simulink model "bms_can_unpack"  (R2026b)
settings: Solver=VariableStepAuto
undefined symbols (not defined in the file or in its folder): Ts
libraries: simulink x16, svdutilitieslib x7
settings Model: Creator=aomar  LastModifiedBy=aomar

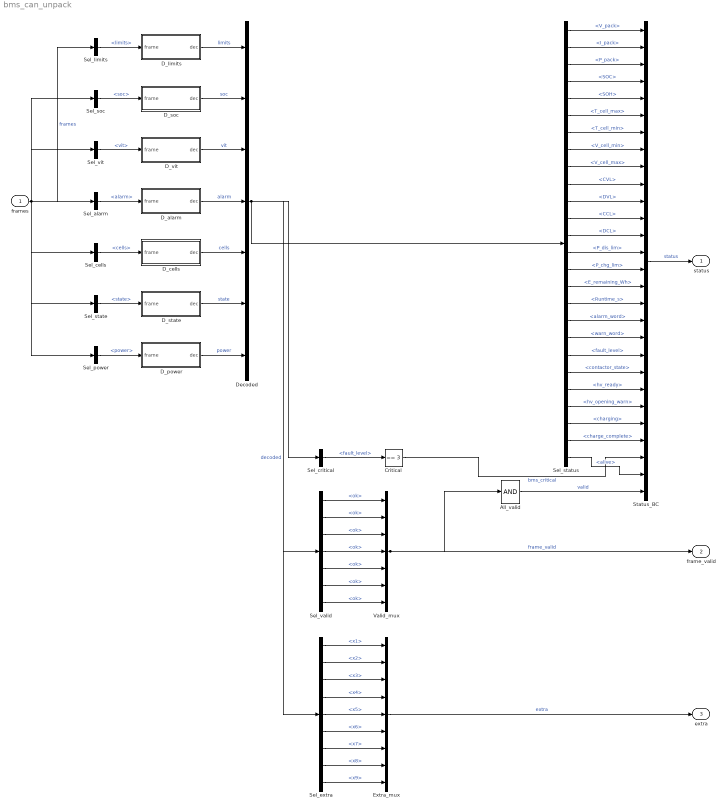
== system bms_can_unpack ==
  frames : Inport  OutDataTypeStr=Bus: Bus_Can1_Bms  SampleTime=Ts.hk
  All_valid : Logic  Inputs=1  AllPortsSameDT=off  OutDataTypeStr=boolean
  Critical : simulink/Logic and Bit Operations/Compare To Constant  relop===  const=3  OutDataTypeStr=boolean
  D_alarm : Subsystem
  D_cells : Subsystem
  D_limits : Subsystem
  D_power : Subsystem
  D_soc : Subsystem
  D_state : Subsystem
  D_vit : Subsystem
  Decoded : BusCreator  Inputs=7
  Extra_mux : Mux  Inputs=9
  Sel_alarm : BusSelector  OutputSignals=alarm
  Sel_cells : BusSelector  OutputSignals=cells
  Sel_critical : BusSelector  OutputSignals=state.fault_level
  Sel_extra : BusSelector  OutputSignals=vit.x1,vit.x2,soc.x3,power.x4,soc.x5,state.x6,state.x7,state.x8,state.x9
  Sel_limits : BusSelector  OutputSignals=limits
  Sel_power : BusSelector  OutputSignals=power
  Sel_soc : BusSelector  OutputSignals=soc
  Sel_state : BusSelector  OutputSignals=state
  Sel_status : BusSelector  OutputSignals=vit.V_pack,vit.I_pack,power.P_pack,soc.SOC,soc.SOH,cells.T_cell_max,cells.T_cell_min,cells.V_cell_min,cells.V_cell_max,limits.CVL,limits.DVL,limits.CCL,limits.DCL,power.P_dis_lim,power.P_chg_lim,state.E_remaining_Wh,state.Runtime_s,alarm.alarm_word,alarm.warn_word,state.fault_level,state.contactor_state,state.hv_ready,state.hv_opening_warn,state.charging,state.charge_complete,state.alive
  Sel_valid : BusSelector  OutputSignals=limits.ok,soc.ok,vit.ok,alarm.ok,cells.ok,state.ok,power.ok
  Sel_vit : BusSelector  OutputSignals=vit
  Status_BC : BusCreator  Inputs=28  OutDataTypeStr=Bus: Bus_BmsStatus  NonVirtualBus=on
      settings: InheritFromInputs=off
  Valid_mux : Mux  Inputs=7
  status : Outport  OutDataTypeStr=Bus: Bus_BmsStatus
  frame_valid : Outport  Port=2  OutDataTypeStr=boolean
  extra : Outport  Port=3  OutDataTypeStr=single
  wires:
  frames/1 -> Sel_limits/1, Sel_power/1, Sel_soc/1, Sel_state/1, Sel_vit/1, Sel_cells/1, Sel_alarm/1  "frames"
  Sel_limits/1 -> D_limits/1(frame)  "<limits>"
  Sel_soc/1 -> D_soc/1(frame)  "<soc>"
  Sel_vit/1 -> D_vit/1(frame)  "<vit>"
  Sel_alarm/1 -> D_alarm/1(frame)  "<alarm>"
  Sel_cells/1 -> D_cells/1(frame)  "<cells>"
  Sel_state/1 -> D_state/1(frame)  "<state>"
  Sel_power/1 -> D_power/1(frame)  "<power>"
  D_limits/1(dec) -> Decoded/1  "limits"
  D_soc/1(dec) -> Decoded/2  "soc"
  D_vit/1(dec) -> Decoded/3  "vit"
  D_alarm/1(dec) -> Decoded/4  "alarm"
  D_cells/1(dec) -> Decoded/5  "cells"
  D_state/1(dec) -> Decoded/6  "state"
  D_power/1(dec) -> Decoded/7  "power"
  Decoded/1 -> Sel_extra/1, Sel_valid/1, Sel_critical/1, Sel_status/1  "decoded"
  Sel_critical/1 -> Critical/1  "<fault_level>"
  Sel_valid/1 -> Valid_mux/1  "<ok>"
  Sel_valid/2 -> Valid_mux/2  "<ok>"
  Sel_valid/3 -> Valid_mux/3  "<ok>"
  Sel_valid/4 -> Valid_mux/4  "<ok>"
  Sel_valid/5 -> Valid_mux/5  "<ok>"
  Sel_valid/6 -> Valid_mux/6  "<ok>"
  Sel_valid/7 -> Valid_mux/7  "<ok>"
  Sel_extra/1 -> Extra_mux/1  "<x1>"
  Sel_extra/2 -> Extra_mux/2  "<x2>"
  Sel_extra/3 -> Extra_mux/3  "<x3>"
  Sel_extra/4 -> Extra_mux/4  "<x4>"
  Sel_extra/5 -> Extra_mux/5  "<x5>"
  Sel_extra/6 -> Extra_mux/6  "<x6>"
  Sel_extra/7 -> Extra_mux/7  "<x7>"
  Sel_extra/8 -> Extra_mux/8  "<x8>"
  Sel_extra/9 -> Extra_mux/9  "<x9>"
  Valid_mux/1 -> All_valid/1, frame_valid/1  "frame_valid"
  Extra_mux/1 -> extra/1  "extra"
  Critical/1 -> Status_BC/26  "bms_critical"
  All_valid/1 -> Status_BC/28  "valid"
  Sel_status/1 -> Status_BC/1  "<V_pack>"
  Sel_status/2 -> Status_BC/2  "<I_pack>"
  Sel_status/3 -> Status_BC/3  "<P_pack>"
  Sel_status/4 -> Status_BC/4  "<SOC>"
  Sel_status/5 -> Status_BC/5  "<SOH>"
  Sel_status/6 -> Status_BC/6  "<T_cell_max>"
  Sel_status/7 -> Status_BC/7  "<T_cell_min>"
  Sel_status/8 -> Status_BC/8  "<V_cell_min>"
  Sel_status/9 -> Status_BC/9  "<V_cell_max>"
  Sel_status/10 -> Status_BC/10  "<CVL>"
  Sel_status/11 -> Status_BC/11  "<DVL>"
  Sel_status/12 -> Status_BC/12  "<CCL>"
  Sel_status/13 -> Status_BC/13  "<DCL>"
  Sel_status/14 -> Status_BC/14  "<P_dis_lim>"
  Sel_status/15 -> Status_BC/15  "<P_chg_lim>"
  Sel_status/16 -> Status_BC/16  "<E_remaining_Wh>"
  Sel_status/17 -> Status_BC/17  "<Runtime_s>"
  Sel_status/18 -> Status_BC/18  "<alarm_word>"
  Sel_status/19 -> Status_BC/19  "<warn_word>"
  Sel_status/20 -> Status_BC/20  "<fault_level>"
  Sel_status/21 -> Status_BC/21  "<contactor_state>"
  Sel_status/22 -> Status_BC/22  "<hv_ready>"
  Sel_status/23 -> Status_BC/23  "<hv_opening_warn>"
  Sel_status/24 -> Status_BC/24  "<charging>"
  Sel_status/25 -> Status_BC/25  "<charge_complete>"
  Sel_status/26 -> Status_BC/27  "<alive>"
  Status_BC/1 -> status/1  "status"

== system bms_can_unpack/D_alarm ==
  frame_id : Inport  PortName=frame  Element=id
  frame_valid : Inport  PortName=frame  Element=valid
  frame_data : Inport  PortName=frame  Element=data
  Decode : Subsystem  TreatAsAtomicUnit=on
  Frame_ok : Logic  AllPortsSameDT=off  OutDataTypeStr=boolean
  ID_match : simulink/Logic and Bit Operations/Compare To Constant  relop===  const=858  OutDataTypeStr=boolean
  dec_ok : Outport  PortName=dec  Element=ok
  dec_alarm_word : Outport  PortName=dec  Element=alarm_word
  dec_warn_word : Outport  PortName=dec  Element=warn_word
  wires:
  frame_id/1 -> ID_match/1  "id"
  ID_match/1 -> Frame_ok/1  "id_match"
  frame_valid/1 -> Frame_ok/2  "valid"
  Frame_ok/1 -> dec_ok/1, Decode/Enable  "frame_ok"
  frame_data/1 -> Decode/1(data)  "data"
  Decode/1(alarm_word) -> dec_alarm_word/1  "alarm_word"
  Decode/2(warn_word) -> dec_warn_word/1  "warn_word"

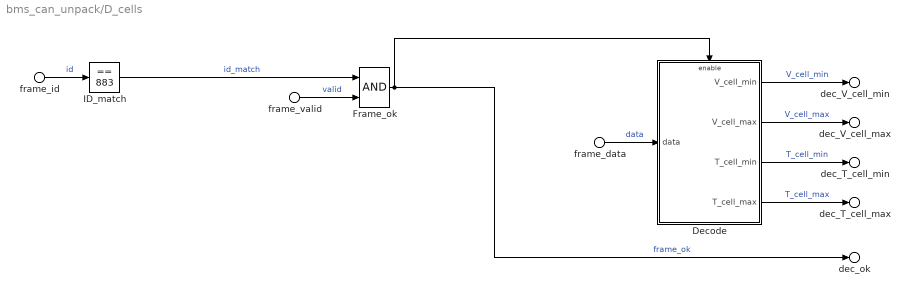
== system bms_can_unpack/D_cells ==
  frame_id : Inport  PortName=frame  Element=id
  frame_valid : Inport  PortName=frame  Element=valid
  frame_data : Inport  PortName=frame  Element=data
  Decode : Subsystem  TreatAsAtomicUnit=on
  Frame_ok : Logic  AllPortsSameDT=off  OutDataTypeStr=boolean
  ID_match : simulink/Logic and Bit Operations/Compare To Constant  relop===  const=883  OutDataTypeStr=boolean
  dec_ok : Outport  PortName=dec  Element=ok
  dec_V_cell_min : Outport  PortName=dec  Element=V_cell_min
  dec_V_cell_max : Outport  PortName=dec  Element=V_cell_max
  dec_T_cell_min : Outport  PortName=dec  Element=T_cell_min
  dec_T_cell_max : Outport  PortName=dec  Element=T_cell_max
  wires:
  frame_id/1 -> ID_match/1  "id"
  ID_match/1 -> Frame_ok/1  "id_match"
  frame_valid/1 -> Frame_ok/2  "valid"
  Frame_ok/1 -> dec_ok/1, Decode/Enable  "frame_ok"
  frame_data/1 -> Decode/1(data)  "data"
  Decode/1(V_cell_min) -> dec_V_cell_min/1  "V_cell_min"
  Decode/2(V_cell_max) -> dec_V_cell_max/1  "V_cell_max"
  Decode/3(T_cell_min) -> dec_T_cell_min/1  "T_cell_min"
  Decode/4(T_cell_max) -> dec_T_cell_max/1  "T_cell_max"

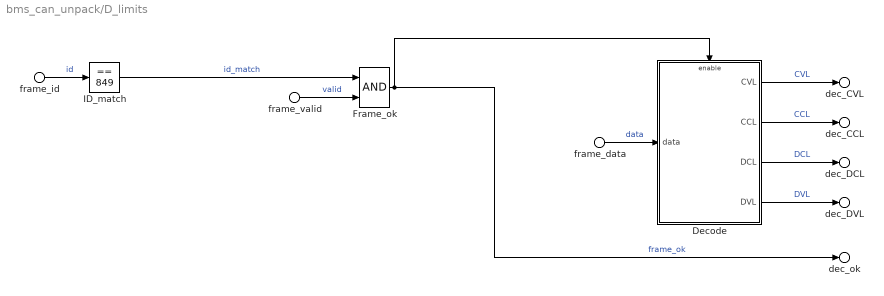
== system bms_can_unpack/D_limits ==
  frame_id : Inport  PortName=frame  Element=id
  frame_valid : Inport  PortName=frame  Element=valid
  frame_data : Inport  PortName=frame  Element=data
  Decode : Subsystem  TreatAsAtomicUnit=on
  Frame_ok : Logic  AllPortsSameDT=off  OutDataTypeStr=boolean
  ID_match : simulink/Logic and Bit Operations/Compare To Constant  relop===  const=849  OutDataTypeStr=boolean
  dec_ok : Outport  PortName=dec  Element=ok
  dec_CVL : Outport  PortName=dec  Element=CVL
  dec_CCL : Outport  PortName=dec  Element=CCL
  dec_DCL : Outport  PortName=dec  Element=DCL
  dec_DVL : Outport  PortName=dec  Element=DVL
  wires:
  frame_id/1 -> ID_match/1  "id"
  ID_match/1 -> Frame_ok/1  "id_match"
  frame_valid/1 -> Frame_ok/2  "valid"
  Frame_ok/1 -> dec_ok/1, Decode/Enable  "frame_ok"
  frame_data/1 -> Decode/1(data)  "data"
  Decode/1(CVL) -> dec_CVL/1  "CVL"
  Decode/2(CCL) -> dec_CCL/1  "CCL"
  Decode/3(DCL) -> dec_DCL/1  "DCL"
  Decode/4(DVL) -> dec_DVL/1  "DVL"

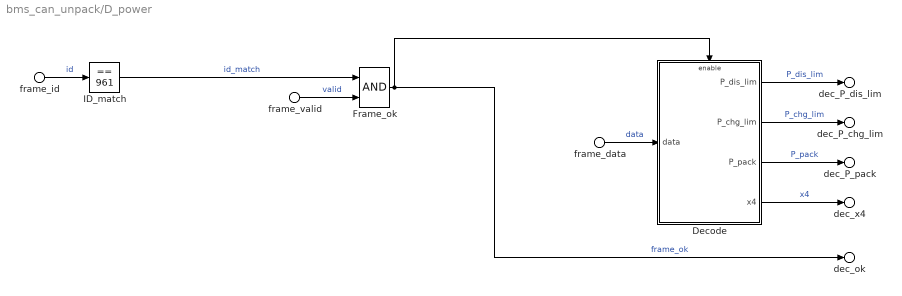
== system bms_can_unpack/D_power ==
  frame_id : Inport  PortName=frame  Element=id
  frame_valid : Inport  PortName=frame  Element=valid
  frame_data : Inport  PortName=frame  Element=data
  Decode : Subsystem  TreatAsAtomicUnit=on
  Frame_ok : Logic  AllPortsSameDT=off  OutDataTypeStr=boolean
  ID_match : simulink/Logic and Bit Operations/Compare To Constant  relop===  const=961  OutDataTypeStr=boolean
  dec_ok : Outport  PortName=dec  Element=ok
  dec_P_dis_lim : Outport  PortName=dec  Element=P_dis_lim
  dec_P_chg_lim : Outport  PortName=dec  Element=P_chg_lim
  dec_P_pack : Outport  PortName=dec  Element=P_pack
  dec_x4 : Outport  PortName=dec  Element=x4
  wires:
  frame_id/1 -> ID_match/1  "id"
  ID_match/1 -> Frame_ok/1  "id_match"
  frame_valid/1 -> Frame_ok/2  "valid"
  Frame_ok/1 -> dec_ok/1, Decode/Enable  "frame_ok"
  frame_data/1 -> Decode/1(data)  "data"
  Decode/1(P_dis_lim) -> dec_P_dis_lim/1  "P_dis_lim"
  Decode/2(P_chg_lim) -> dec_P_chg_lim/1  "P_chg_lim"
  Decode/3(P_pack) -> dec_P_pack/1  "P_pack"
  Decode/4(x4) -> dec_x4/1  "x4"

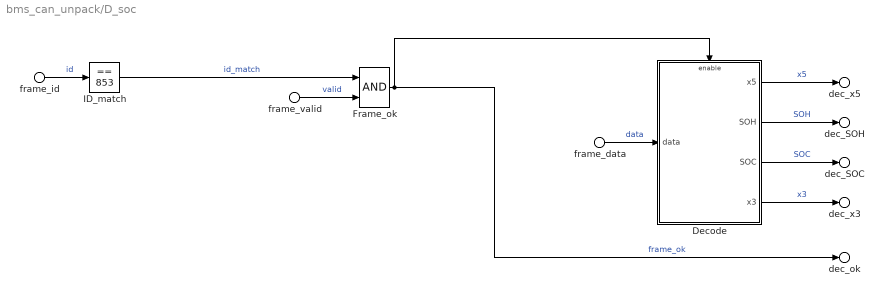
== system bms_can_unpack/D_soc ==
  frame_id : Inport  PortName=frame  Element=id
  frame_valid : Inport  PortName=frame  Element=valid
  frame_data : Inport  PortName=frame  Element=data
  Decode : Subsystem  TreatAsAtomicUnit=on
  Frame_ok : Logic  AllPortsSameDT=off  OutDataTypeStr=boolean
  ID_match : simulink/Logic and Bit Operations/Compare To Constant  relop===  const=853  OutDataTypeStr=boolean
  dec_ok : Outport  PortName=dec  Element=ok
  dec_x5 : Outport  PortName=dec  Element=x5
  dec_SOH : Outport  PortName=dec  Element=SOH
  dec_SOC : Outport  PortName=dec  Element=SOC
  dec_x3 : Outport  PortName=dec  Element=x3
  wires:
  frame_id/1 -> ID_match/1  "id"
  ID_match/1 -> Frame_ok/1  "id_match"
  frame_valid/1 -> Frame_ok/2  "valid"
  Frame_ok/1 -> dec_ok/1, Decode/Enable  "frame_ok"
  frame_data/1 -> Decode/1(data)  "data"
  Decode/1(x5) -> dec_x5/1  "x5"
  Decode/2(SOH) -> dec_SOH/1  "SOH"
  Decode/3(SOC) -> dec_SOC/1  "SOC"
  Decode/4(x3) -> dec_x3/1  "x3"

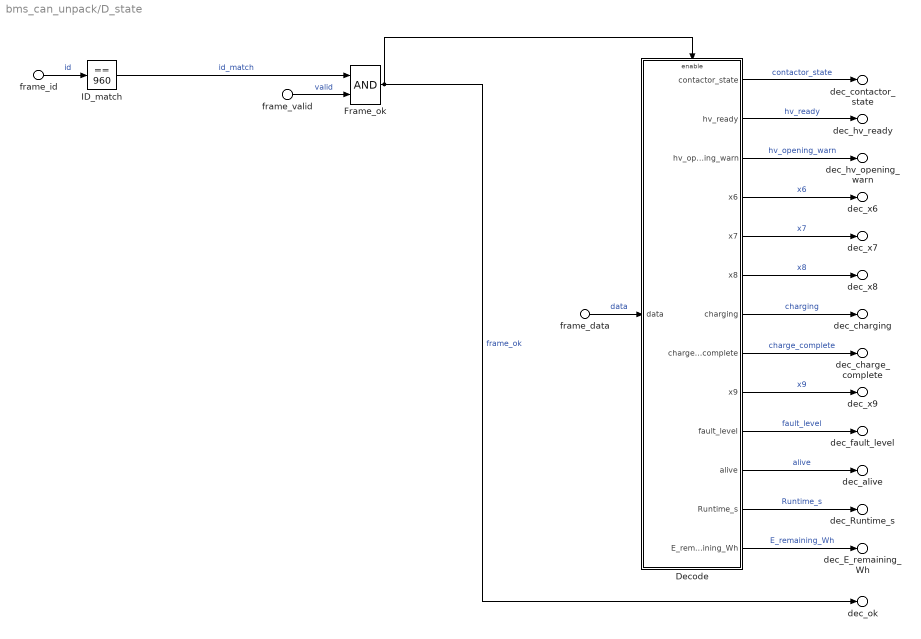
== system bms_can_unpack/D_state ==
  frame_id : Inport  PortName=frame  Element=id
  frame_valid : Inport  PortName=frame  Element=valid
  frame_data : Inport  PortName=frame  Element=data
  Decode : Subsystem  TreatAsAtomicUnit=on
  Frame_ok : Logic  AllPortsSameDT=off  OutDataTypeStr=boolean
  ID_match : simulink/Logic and Bit Operations/Compare To Constant  relop===  const=960  OutDataTypeStr=boolean
  dec_ok : Outport  PortName=dec  Element=ok
  dec_contactor_state : Outport  PortName=dec  Element=contactor_state
  dec_hv_ready : Outport  PortName=dec  Element=hv_ready
  dec_hv_opening_warn : Outport  PortName=dec  Element=hv_opening_warn
  dec_x6 : Outport  PortName=dec  Element=x6
  dec_x7 : Outport  PortName=dec  Element=x7
  dec_x8 : Outport  PortName=dec  Element=x8
  dec_charging : Outport  PortName=dec  Element=charging
  dec_charge_complete : Outport  PortName=dec  Element=charge_complete
  dec_x9 : Outport  PortName=dec  Element=x9
  dec_fault_level : Outport  PortName=dec  Element=fault_level
  dec_alive : Outport  PortName=dec  Element=alive
  dec_Runtime_s : Outport  PortName=dec  Element=Runtime_s
  dec_E_remaining_Wh : Outport  PortName=dec  Element=E_remaining_Wh
  wires:
  frame_id/1 -> ID_match/1  "id"
  ID_match/1 -> Frame_ok/1  "id_match"
  frame_valid/1 -> Frame_ok/2  "valid"
  Frame_ok/1 -> dec_ok/1, Decode/Enable  "frame_ok"
  frame_data/1 -> Decode/1(data)  "data"
  Decode/1(contactor_state) -> dec_contactor_state/1  "contactor_state"
  Decode/2(hv_ready) -> dec_hv_ready/1  "hv_ready"
  Decode/3(hv_opening_warn) -> dec_hv_opening_warn/1  "hv_opening_warn"
  Decode/4(x6) -> dec_x6/1  "x6"
  Decode/5(x7) -> dec_x7/1  "x7"
  Decode/6(x8) -> dec_x8/1  "x8"
  Decode/7(charging) -> dec_charging/1  "charging"
  Decode/8(charge_complete) -> dec_charge_complete/1  "charge_complete"
  Decode/9(x9) -> dec_x9/1  "x9"
  Decode/10(fault_level) -> dec_fault_level/1  "fault_level"
  Decode/11(alive) -> dec_alive/1  "alive"
  Decode/12(Runtime_s) -> dec_Runtime_s/1  "Runtime_s"
  Decode/13(E_remaining_Wh) -> dec_E_remaining_Wh/1  "E_remaining_Wh"

== system bms_can_unpack/D_vit ==
  frame_id : Inport  PortName=frame  Element=id
  frame_valid : Inport  PortName=frame  Element=valid
  frame_data : Inport  PortName=frame  Element=data
  Decode : Subsystem  TreatAsAtomicUnit=on
  Frame_ok : Logic  AllPortsSameDT=off  OutDataTypeStr=boolean
  ID_match : simulink/Logic and Bit Operations/Compare To Constant  relop===  const=854  OutDataTypeStr=boolean
  dec_ok : Outport  PortName=dec  Element=ok
  dec_V_pack : Outport  PortName=dec  Element=V_pack
  dec_I_pack : Outport  PortName=dec  Element=I_pack
  dec_x2 : Outport  PortName=dec  Element=x2
  dec_x1 : Outport  PortName=dec  Element=x1
  wires:
  frame_id/1 -> ID_match/1  "id"
  ID_match/1 -> Frame_ok/1  "id_match"
  frame_valid/1 -> Frame_ok/2  "valid"
  Frame_ok/1 -> dec_ok/1, Decode/Enable  "frame_ok"
  frame_data/1 -> Decode/1(data)  "data"
  Decode/1(V_pack) -> dec_V_pack/1  "V_pack"
  Decode/2(I_pack) -> dec_I_pack/1  "I_pack"
  Decode/3(x2) -> dec_x2/1  "x2"
  Decode/4(x1) -> dec_x1/1  "x1"

== system bms_can_unpack/D_alarm/Decode ==
  data : Inport
  Enable : EnablePort
  Unpack : svdutilitieslib/Byte Unpack  dimensions={1,1}  datatypes={'uint32','uint32'}  byteAlign=1  blockPlatform=arduinoert
      settings: LibrarySourceBlock=mcblib/Signal Management/Byte Unpack
  f1 : DataTypeConversion  OutDataTypeStr=uint32  SaturateOnIntegerOverflow=off  RndMeth=Floor
  f2 : DataTypeConversion  OutDataTypeStr=uint32  SaturateOnIntegerOverflow=off  RndMeth=Floor
  alarm_word : Outport  InitialOutput=0
  warn_word : Outport  Port=2  InitialOutput=0
  wires:
  data/1 -> Unpack/1  "data"
  Unpack/1 -> f1/1  "Unpack_1"
  Unpack/2 -> f2/1  "Unpack_2"
  f1/1 -> alarm_word/1  "alarm_word"
  f2/1 -> warn_word/1  "warn_word"

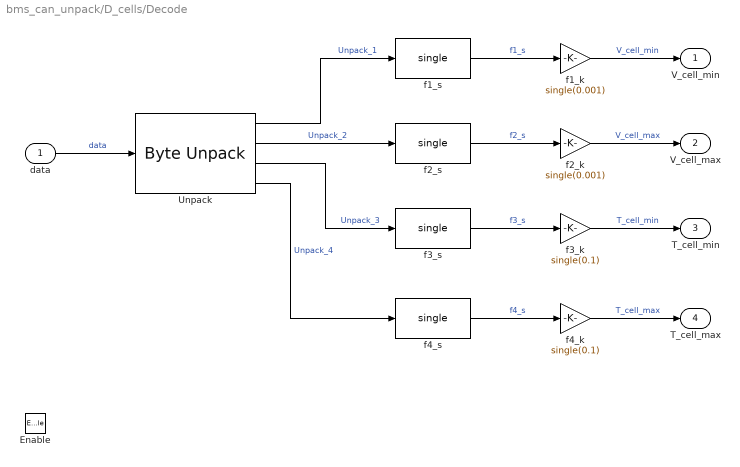
== system bms_can_unpack/D_cells/Decode ==
  data : Inport
  Enable : EnablePort
  Unpack : svdutilitieslib/Byte Unpack  dimensions={1,1,1,1}  datatypes={'uint16','uint16','uint16','uint16'}  byteAlign=1  blockPlatform=arduinoert
      settings: LibrarySourceBlock=mcblib/Signal Management/Byte Unpack
  f1_k : Gain  Gain=single(0.001)
  f1_s : DataTypeConversion  OutDataTypeStr=single  SaturateOnIntegerOverflow=off  RndMeth=Floor
  f2_k : Gain  Gain=single(0.001)
  f2_s : DataTypeConversion  OutDataTypeStr=single  SaturateOnIntegerOverflow=off  RndMeth=Floor
  f3_k : Gain  Gain=single(0.1)
  f3_s : DataTypeConversion  OutDataTypeStr=single  SaturateOnIntegerOverflow=off  RndMeth=Floor
  f4_k : Gain  Gain=single(0.1)
  f4_s : DataTypeConversion  OutDataTypeStr=single  SaturateOnIntegerOverflow=off  RndMeth=Floor
  V_cell_min : Outport  InitialOutput=0
  V_cell_max : Outport  Port=2  InitialOutput=0
  T_cell_min : Outport  Port=3  InitialOutput=0
  T_cell_max : Outport  Port=4  InitialOutput=0
  wires:
  data/1 -> Unpack/1  "data"
  Unpack/1 -> f1_s/1  "Unpack_1"
  Unpack/2 -> f2_s/1  "Unpack_2"
  Unpack/3 -> f3_s/1  "Unpack_3"
  Unpack/4 -> f4_s/1  "Unpack_4"
  f1_s/1 -> f1_k/1  "f1_s"
  f2_s/1 -> f2_k/1  "f2_s"
  f3_s/1 -> f3_k/1  "f3_s"
  f4_s/1 -> f4_k/1  "f4_s"
  f1_k/1 -> V_cell_min/1  "V_cell_min"
  f2_k/1 -> V_cell_max/1  "V_cell_max"
  f3_k/1 -> T_cell_min/1  "T_cell_min"
  f4_k/1 -> T_cell_max/1  "T_cell_max"

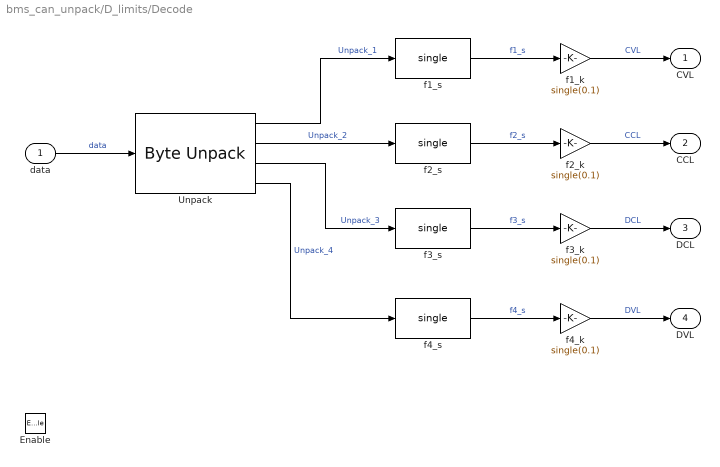
== system bms_can_unpack/D_limits/Decode ==
  data : Inport
  Enable : EnablePort
  Unpack : svdutilitieslib/Byte Unpack  dimensions={1,1,1,1}  datatypes={'uint16','int16','int16','uint16'}  byteAlign=1  blockPlatform=arduinoert
      settings: LibrarySourceBlock=mcblib/Signal Management/Byte Unpack
  f1_k : Gain  Gain=single(0.1)
  f1_s : DataTypeConversion  OutDataTypeStr=single  SaturateOnIntegerOverflow=off  RndMeth=Floor
  f2_k : Gain  Gain=single(0.1)
  f2_s : DataTypeConversion  OutDataTypeStr=single  SaturateOnIntegerOverflow=off  RndMeth=Floor
  f3_k : Gain  Gain=single(0.1)
  f3_s : DataTypeConversion  OutDataTypeStr=single  SaturateOnIntegerOverflow=off  RndMeth=Floor
  f4_k : Gain  Gain=single(0.1)
  f4_s : DataTypeConversion  OutDataTypeStr=single  SaturateOnIntegerOverflow=off  RndMeth=Floor
  CVL : Outport  InitialOutput=0
  CCL : Outport  Port=2  InitialOutput=0
  DCL : Outport  Port=3  InitialOutput=0
  DVL : Outport  Port=4  InitialOutput=0
  wires:
  data/1 -> Unpack/1  "data"
  Unpack/1 -> f1_s/1  "Unpack_1"
  Unpack/2 -> f2_s/1  "Unpack_2"
  Unpack/3 -> f3_s/1  "Unpack_3"
  Unpack/4 -> f4_s/1  "Unpack_4"
  f1_s/1 -> f1_k/1  "f1_s"
  f2_s/1 -> f2_k/1  "f2_s"
  f3_s/1 -> f3_k/1  "f3_s"
  f4_s/1 -> f4_k/1  "f4_s"
  f1_k/1 -> CVL/1  "CVL"
  f2_k/1 -> CCL/1  "CCL"
  f3_k/1 -> DCL/1  "DCL"
  f4_k/1 -> DVL/1  "DVL"

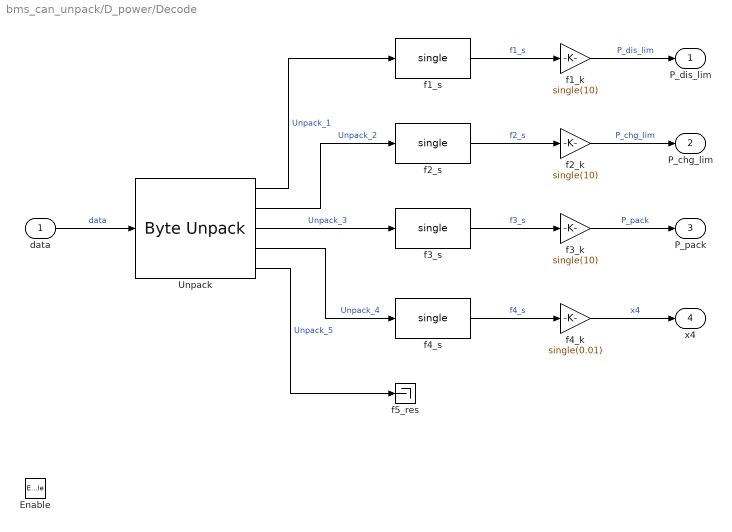
== system bms_can_unpack/D_power/Decode ==
  data : Inport
  Enable : EnablePort
  Unpack : svdutilitieslib/Byte Unpack  dimensions={1,1,1,1,1}  datatypes={'uint16','uint16','int16','uint8','uint8'}  byteAlign=1  blockPlatform=arduinoert
      settings: LibrarySourceBlock=mcblib/Signal Management/Byte Unpack
  f1_k : Gain  Gain=single(10)
  f1_s : DataTypeConversion  OutDataTypeStr=single  SaturateOnIntegerOverflow=off  RndMeth=Floor
  f2_k : Gain  Gain=single(10)
  f2_s : DataTypeConversion  OutDataTypeStr=single  SaturateOnIntegerOverflow=off  RndMeth=Floor
  f3_k : Gain  Gain=single(10)
  f3_s : DataTypeConversion  OutDataTypeStr=single  SaturateOnIntegerOverflow=off  RndMeth=Floor
  f4_k : Gain  Gain=single(0.01)
  f4_s : DataTypeConversion  OutDataTypeStr=single  SaturateOnIntegerOverflow=off  RndMeth=Floor
  f5_res : Terminator
  P_dis_lim : Outport  InitialOutput=0
  P_chg_lim : Outport  Port=2  InitialOutput=0
  P_pack : Outport  Port=3  InitialOutput=0
  x4 : Outport  Port=4  InitialOutput=0
  wires:
  data/1 -> Unpack/1  "data"
  Unpack/1 -> f1_s/1  "Unpack_1"
  Unpack/2 -> f2_s/1  "Unpack_2"
  Unpack/3 -> f3_s/1  "Unpack_3"
  Unpack/4 -> f4_s/1  "Unpack_4"
  Unpack/5 -> f5_res/1  "Unpack_5"
  f1_s/1 -> f1_k/1  "f1_s"
  f2_s/1 -> f2_k/1  "f2_s"
  f3_s/1 -> f3_k/1  "f3_s"
  f4_s/1 -> f4_k/1  "f4_s"
  f1_k/1 -> P_dis_lim/1  "P_dis_lim"
  f2_k/1 -> P_chg_lim/1  "P_chg_lim"
  f3_k/1 -> P_pack/1  "P_pack"
  f4_k/1 -> x4/1  "x4"

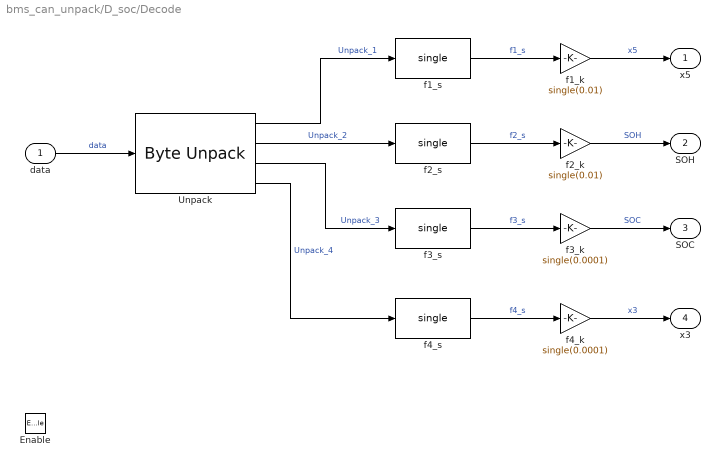
== system bms_can_unpack/D_soc/Decode ==
  data : Inport
  Enable : EnablePort
  Unpack : svdutilitieslib/Byte Unpack  dimensions={1,1,1,1}  datatypes={'uint16','uint16','uint16','uint16'}  byteAlign=1  blockPlatform=arduinoert
      settings: LibrarySourceBlock=mcblib/Signal Management/Byte Unpack
  f1_k : Gain  Gain=single(0.01)
  f1_s : DataTypeConversion  OutDataTypeStr=single  SaturateOnIntegerOverflow=off  RndMeth=Floor
  f2_k : Gain  Gain=single(0.01)
  f2_s : DataTypeConversion  OutDataTypeStr=single  SaturateOnIntegerOverflow=off  RndMeth=Floor
  f3_k : Gain  Gain=single(0.0001)
  f3_s : DataTypeConversion  OutDataTypeStr=single  SaturateOnIntegerOverflow=off  RndMeth=Floor
  f4_k : Gain  Gain=single(0.0001)
  f4_s : DataTypeConversion  OutDataTypeStr=single  SaturateOnIntegerOverflow=off  RndMeth=Floor
  x5 : Outport  InitialOutput=0
  SOH : Outport  Port=2  InitialOutput=0
  SOC : Outport  Port=3  InitialOutput=0
  x3 : Outport  Port=4  InitialOutput=0
  wires:
  data/1 -> Unpack/1  "data"
  Unpack/1 -> f1_s/1  "Unpack_1"
  Unpack/2 -> f2_s/1  "Unpack_2"
  Unpack/3 -> f3_s/1  "Unpack_3"
  Unpack/4 -> f4_s/1  "Unpack_4"
  f1_s/1 -> f1_k/1  "f1_s"
  f2_s/1 -> f2_k/1  "f2_s"
  f3_s/1 -> f3_k/1  "f3_s"
  f4_s/1 -> f4_k/1  "f4_s"
  f1_k/1 -> x5/1  "x5"
  f2_k/1 -> SOH/1  "SOH"
  f3_k/1 -> SOC/1  "SOC"
  f4_k/1 -> x3/1  "x3"

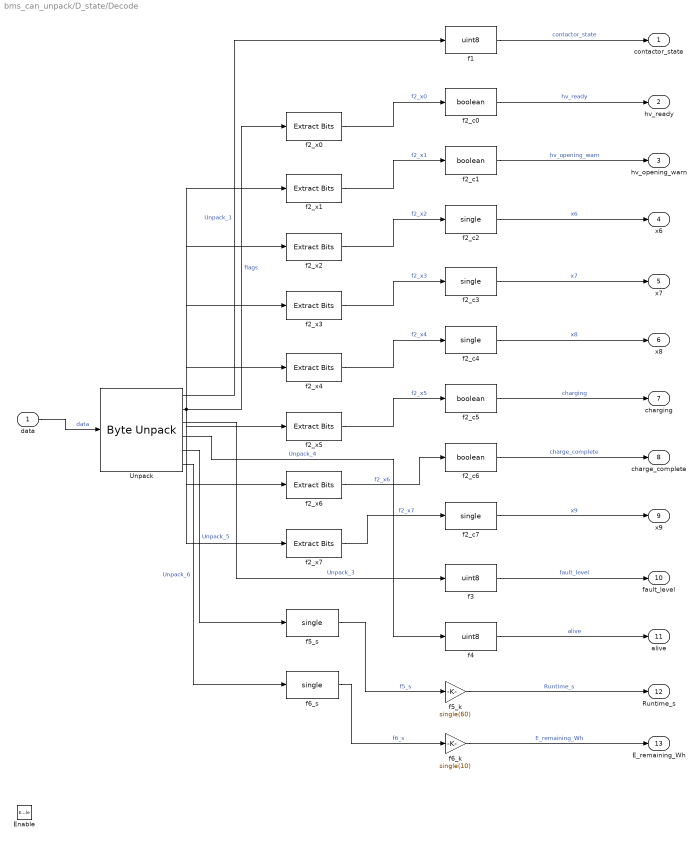
== system bms_can_unpack/D_state/Decode ==
  data : Inport
  Enable : EnablePort
  Unpack : svdutilitieslib/Byte Unpack  dimensions={1,1,1,1,1,1}  datatypes={'uint8','uint8','uint8','uint8','uint16','uint16'}  byteAlign=1  blockPlatform=arduinoert
      settings: LibrarySourceBlock=mcblib/Signal Management/Byte Unpack
  f1 : DataTypeConversion  OutDataTypeStr=uint8  SaturateOnIntegerOverflow=off  RndMeth=Floor
  f2_c{0..1,5..6} (4 alike) : DataTypeConversion  OutDataTypeStr=boolean  SaturateOnIntegerOverflow=off  RndMeth=Floor
  f2_c{2..4,7} (4 alike) : DataTypeConversion  OutDataTypeStr=single  SaturateOnIntegerOverflow=off  RndMeth=Floor
  f2_x0 : simulink/Logic and Bit Operations/Extract Bits  bitsToExtract=Range of bits  numBits=8  bitIdxRange=[0 0]  outScalingMode=Treat bit field as an integer
  f2_x1 : simulink/Logic and Bit Operations/Extract Bits  bitsToExtract=Range of bits  numBits=8  bitIdxRange=[1 1]  outScalingMode=Treat bit field as an integer
  f2_x2 : simulink/Logic and Bit Operations/Extract Bits  bitsToExtract=Range of bits  numBits=8  bitIdxRange=[2 2]  outScalingMode=Treat bit field as an integer
  f2_x3 : simulink/Logic and Bit Operations/Extract Bits  bitsToExtract=Range of bits  numBits=8  bitIdxRange=[3 3]  outScalingMode=Treat bit field as an integer
  f2_x4 : simulink/Logic and Bit Operations/Extract Bits  bitsToExtract=Range of bits  numBits=8  bitIdxRange=[4 4]  outScalingMode=Treat bit field as an integer
  f2_x5 : simulink/Logic and Bit Operations/Extract Bits  bitsToExtract=Range of bits  numBits=8  bitIdxRange=[5 5]  outScalingMode=Treat bit field as an integer
  f2_x6 : simulink/Logic and Bit Operations/Extract Bits  bitsToExtract=Range of bits  numBits=8  bitIdxRange=[6 6]  outScalingMode=Treat bit field as an integer
  f2_x7 : simulink/Logic and Bit Operations/Extract Bits  bitsToExtract=Range of bits  numBits=8  bitIdxRange=[7 7]  outScalingMode=Treat bit field as an integer
  f3 : DataTypeConversion  OutDataTypeStr=uint8  SaturateOnIntegerOverflow=off  RndMeth=Floor
  f4 : DataTypeConversion  OutDataTypeStr=uint8  SaturateOnIntegerOverflow=off  RndMeth=Floor
  f5_k : Gain  Gain=single(60)
  f5_s : DataTypeConversion  OutDataTypeStr=single  SaturateOnIntegerOverflow=off  RndMeth=Floor
  f6_k : Gain  Gain=single(10)
  f6_s : DataTypeConversion  OutDataTypeStr=single  SaturateOnIntegerOverflow=off  RndMeth=Floor
  contactor_state : Outport  InitialOutput=0
  hv_ready : Outport  Port=2  InitialOutput=0
  hv_opening_warn : Outport  Port=3  InitialOutput=0
  x6 : Outport  Port=4  InitialOutput=0
  x7 : Outport  Port=5  InitialOutput=0
  x8 : Outport  Port=6  InitialOutput=0
  charging : Outport  Port=7  InitialOutput=0
  charge_complete : Outport  Port=8  InitialOutput=0
  x9 : Outport  Port=9  InitialOutput=0
  fault_level : Outport  Port=10  InitialOutput=0
  alive : Outport  Port=11  InitialOutput=0
  Runtime_s : Outport  Port=12  InitialOutput=0
  E_remaining_Wh : Outport  Port=13  InitialOutput=0
  wires:
  data/1 -> Unpack/1  "data"
  Unpack/1 -> f1/1  "Unpack_1"
  Unpack/2 -> f2_x0/1, f2_x1/1, f2_x2/1, f2_x7/1, f2_x3/1, f2_x6/1, f2_x4/1, f2_x5/1  "flags"
  Unpack/3 -> f3/1  "Unpack_3"
  Unpack/4 -> f4/1  "Unpack_4"
  Unpack/5 -> f5_s/1  "Unpack_5"
  Unpack/6 -> f6_s/1  "Unpack_6"
  f5_s/1 -> f5_k/1  "f5_s"
  f6_s/1 -> f6_k/1  "f6_s"
  f2_x0/1 -> f2_c0/1  "f2_x0"
  f2_x1/1 -> f2_c1/1  "f2_x1"
  f2_x2/1 -> f2_c2/1  "f2_x2"
  f2_x3/1 -> f2_c3/1  "f2_x3"
  f2_x4/1 -> f2_c4/1  "f2_x4"
  f2_x5/1 -> f2_c5/1  "f2_x5"
  f2_x6/1 -> f2_c6/1  "f2_x6"
  f2_x7/1 -> f2_c7/1  "f2_x7"
  f5_k/1 -> Runtime_s/1  "Runtime_s"
  f6_k/1 -> E_remaining_Wh/1  "E_remaining_Wh"
  f1/1 -> contactor_state/1  "contactor_state"
  f2_c0/1 -> hv_ready/1  "hv_ready"
  f2_c1/1 -> hv_opening_warn/1  "hv_opening_warn"
  f2_c2/1 -> x6/1  "x6"
  f2_c3/1 -> x7/1  "x7"
  f2_c4/1 -> x8/1  "x8"
  f2_c5/1 -> charging/1  "charging"
  f2_c6/1 -> charge_complete/1  "charge_complete"
  f2_c7/1 -> x9/1  "x9"
  f3/1 -> fault_level/1  "fault_level"
  f4/1 -> alive/1  "alive"

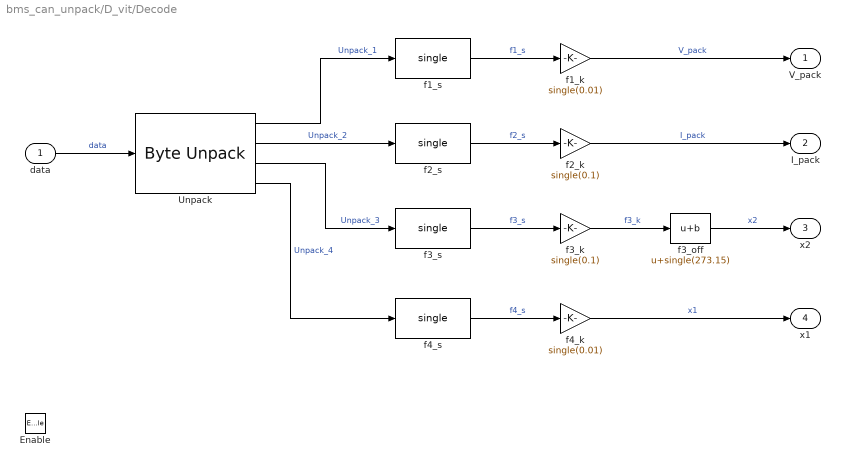
== system bms_can_unpack/D_vit/Decode ==
  data : Inport
  Enable : EnablePort
  Unpack : svdutilitieslib/Byte Unpack  dimensions={1,1,1,1}  datatypes={'int16','int16','int16','uint16'}  byteAlign=1  blockPlatform=arduinoert
      settings: LibrarySourceBlock=mcblib/Signal Management/Byte Unpack
  f1_k : Gain  Gain=single(0.01)
  f1_s : DataTypeConversion  OutDataTypeStr=single  SaturateOnIntegerOverflow=off  RndMeth=Floor
  f2_k : Gain  Gain=single(0.1)
  f2_s : DataTypeConversion  OutDataTypeStr=single  SaturateOnIntegerOverflow=off  RndMeth=Floor
  f3_k : Gain  Gain=single(0.1)
  f3_off : Bias  Bias=single(273.15)  SaturateOnIntegerOverflow=off
  f3_s : DataTypeConversion  OutDataTypeStr=single  SaturateOnIntegerOverflow=off  RndMeth=Floor
  f4_k : Gain  Gain=single(0.01)
  f4_s : DataTypeConversion  OutDataTypeStr=single  SaturateOnIntegerOverflow=off  RndMeth=Floor
  V_pack : Outport  InitialOutput=0
  I_pack : Outport  Port=2  InitialOutput=0
  x2 : Outport  Port=3  InitialOutput=0
  x1 : Outport  Port=4  InitialOutput=0
  wires:
  data/1 -> Unpack/1  "data"
  Unpack/1 -> f1_s/1  "Unpack_1"
  Unpack/2 -> f2_s/1  "Unpack_2"
  Unpack/3 -> f3_s/1  "Unpack_3"
  Unpack/4 -> f4_s/1  "Unpack_4"
  f1_s/1 -> f1_k/1  "f1_s"
  f2_s/1 -> f2_k/1  "f2_s"
  f3_s/1 -> f3_k/1  "f3_s"
  f4_s/1 -> f4_k/1  "f4_s"
  f1_k/1 -> V_pack/1  "V_pack"
  f2_k/1 -> I_pack/1  "I_pack"
  f3_k/1 -> f3_off/1  "f3_k"
  f4_k/1 -> x1/1  "x1"
  f3_off/1 -> x2/1  "x2"
